simulink model "Electronics_Plant"  (R2026b)
settings: Solver=VariableStepAuto
undefined symbols (not defined in the file or in its folder): P, Ts
settings Model: Creator=aomar  LastModifiedBy=aomar

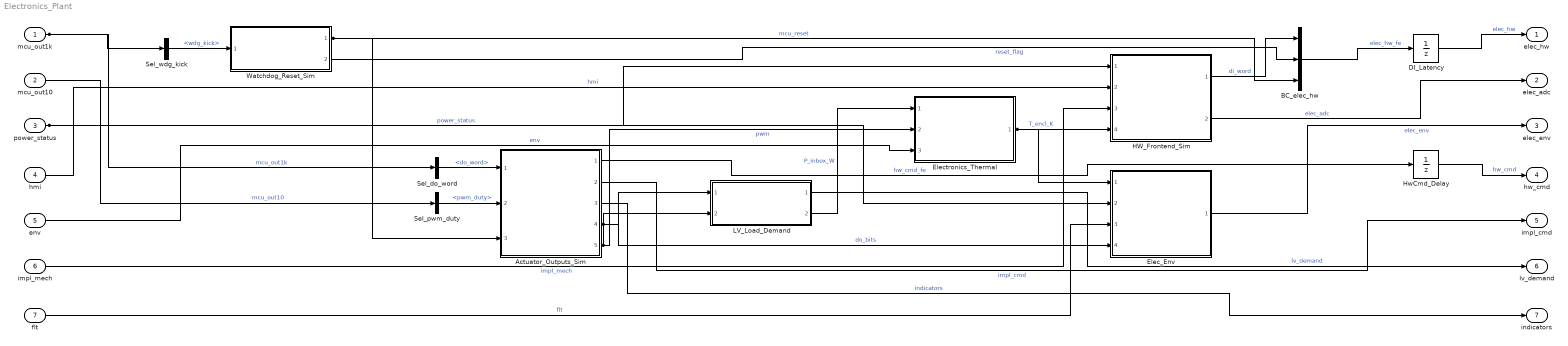
== system Electronics_Plant ==
  mcu_out1k : Inport  OutDataTypeStr=Bus: Bus_McuOut1k  SampleTime=Ts.base
  mcu_out10 : Inport  Port=2  OutDataTypeStr=Bus: Bus_McuOut10  SampleTime=Ts.ctrl
  power_status : Inport  Port=3  OutDataTypeStr=Bus: Bus_PowerStatus  SampleTime=Ts.base
  hmi : Inport  Port=4  OutDataTypeStr=Bus: Bus_HmiInputs  SampleTime=Ts.base
  env : Inport  Port=5  OutDataTypeStr=Bus: Bus_EnvState  SampleTime=Ts.hk
  impl_mech : Inport  Port=6  OutDataTypeStr=Bus: Bus_ImplMechState  SampleTime=Ts.ctrl
  flt : Inport  Port=7  OutDataTypeStr=Bus: Bus_FaultInject  SampleTime=Ts.base
  Actuator_Outputs_Sim : Subsystem  ReferencedSubsystem=elp_actuators
  BC_elec_hw : BusCreator  Inputs=3  OutDataTypeStr=Bus: Bus_ElecHwIn  NonVirtualBus=on
      settings: InheritFromInputs=off
  DI_Latency : UnitDelay  InitialCondition=P.ic.Bus_ElecHwIn  SampleTime=Ts.base
  Elec_Env : Subsystem  ReferencedSubsystem=elp_elec_env
  Electronics_Thermal : Subsystem  ReferencedSubsystem=elp_thermal
  HW_Frontend_Sim : Subsystem  ReferencedSubsystem=elp_hw_frontend
  HwCmd_Delay : UnitDelay  InitialCondition=P.ic.Bus_PowerHwCmd  SampleTime=Ts.base
  LV_Load_Demand : Subsystem  ReferencedSubsystem=elp_lv_demand
  Sel_do_word : BusSelector  OutputSignals=do_word
  Sel_pwm_duty : BusSelector  OutputSignals=pwm_duty
  Sel_wdg_kick : BusSelector  OutputSignals=wdg_kick
  Watchdog_Reset_Sim : Subsystem  ReferencedSubsystem=elp_watchdog_reset
  elec_hw : Outport  OutDataTypeStr=Bus: Bus_ElecHwIn
  elec_adc : Outport  Port=2  OutDataTypeStr=Bus: Bus_ElecAdc
  elec_env : Outport  Port=3  OutDataTypeStr=Bus: Bus_ElecEnv
  hw_cmd : Outport  Port=4  OutDataTypeStr=Bus: Bus_PowerHwCmd
  impl_cmd : Outport  Port=5  OutDataTypeStr=Bus: Bus_ImplementCmd
  lv_demand : Outport  Port=6  OutDataTypeStr=Bus: Bus_LV_LoadDemand
  indicators : Outport  Port=7  OutDataTypeStr=Bus: Bus_IndicatorOut
  wires:
  mcu_out1k/1 -> Sel_do_word/1, Sel_wdg_kick/1  "mcu_out1k"
  mcu_out10/1 -> Sel_pwm_duty/1  "mcu_out10"
  power_status/1 -> Elec_Env/2, HW_Frontend_Sim/1  "power_status"
  hmi/1 -> HW_Frontend_Sim/2  "hmi"
  env/1 -> Electronics_Thermal/3  "env"
  impl_mech/1 -> HW_Frontend_Sim/3  "impl_mech"
  flt/1 -> Elec_Env/3  "flt"
  Sel_wdg_kick/1 -> Watchdog_Reset_Sim/1  "<wdg_kick>"
  Watchdog_Reset_Sim/1 -> Actuator_Outputs_Sim/3, BC_elec_hw/3  "mcu_reset"
  Watchdog_Reset_Sim/2 -> BC_elec_hw/2  "reset_flag"
  Sel_do_word/1 -> Actuator_Outputs_Sim/1  "<do_word>"
  Sel_pwm_duty/1 -> Actuator_Outputs_Sim/2  "<pwm_duty>"
  Actuator_Outputs_Sim/1 -> HwCmd_Delay/1  "hw_cmd_fe"
  Actuator_Outputs_Sim/2 -> impl_cmd/1  "impl_cmd"
  Actuator_Outputs_Sim/3 -> indicators/1  "indicators"
  LV_Load_Demand/1 -> lv_demand/1  "lv_demand"
  LV_Load_Demand/2 -> Electronics_Thermal/1  "P_inbox_W"
  Electronics_Thermal/1 -> Elec_Env/1, HW_Frontend_Sim/4  "T_encl_K"
  HW_Frontend_Sim/1 -> BC_elec_hw/1  "di_word"
  HW_Frontend_Sim/2 -> elec_adc/1  "elec_adc"
  Elec_Env/1 -> elec_env/1  "elec_env"
  BC_elec_hw/1 -> DI_Latency/1  "elec_hw_fe"
  DI_Latency/1 -> elec_hw/1  "elec_hw"
  HwCmd_Delay/1 -> hw_cmd/1  "hw_cmd"
  Actuator_Outputs_Sim/4 -> LV_Load_Demand/1, Elec_Env/4  "do_bits"
  Actuator_Outputs_Sim/5 -> Electronics_Thermal/2, LV_Load_Demand/2  "pwm"
